simulink model "MomentEquation"  (R2024b)
settings: Solver=ode4  StartTime=0.0  StopTime=10  FixedStep=0.001  RelTol=1e-3
PreLoadFcn:
  | run UAVProperty
values from neighbouring files (symbols this model uses):
  I = [Ixx Ixy Ixz ... (first row only)    [UAVProperty.m]    (also in UnmannedAerialVehicle.m)
libraries: simulink x3, shared6dof x1, matrix_library x1
settings Model: Creator=LocoalKOH  LastModifiedBy=LocoalKOH

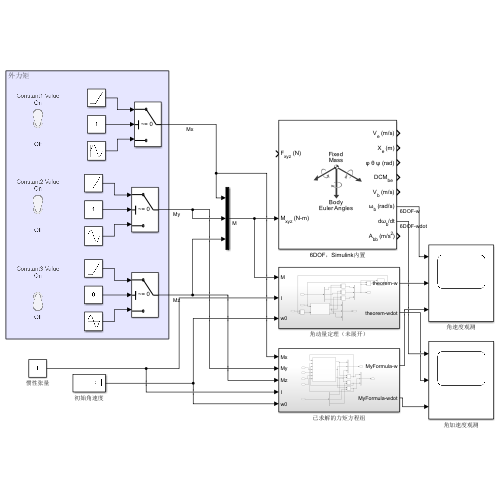
[thumbnail: Simulink's stored preview of the top-level diagram]
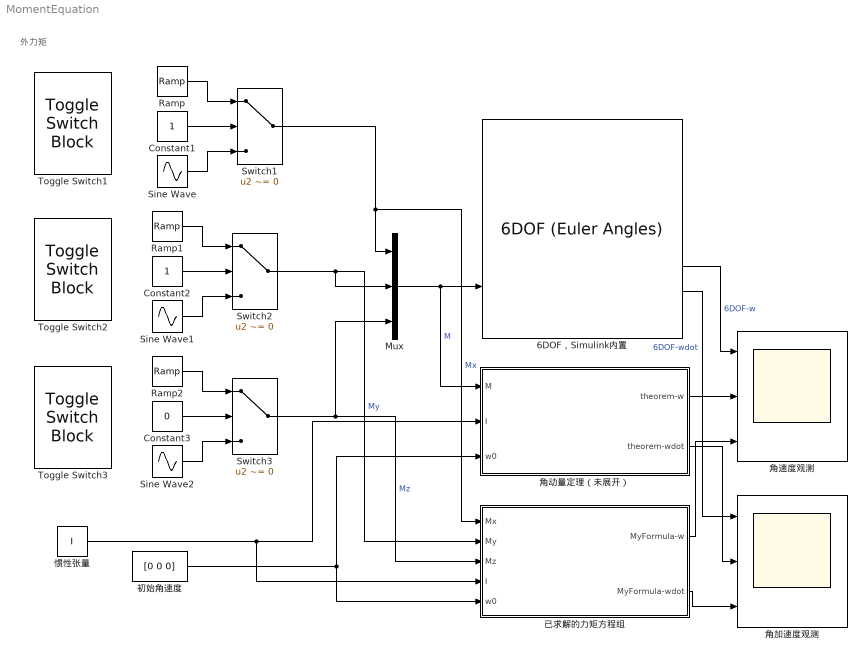
== system MomentEquation ==
  note: 外力矩
  6DOF，Simulink内置 : shared6dof/6DOF (Euler Angles)  units=Metric (MKS)  mtype=Fixed  rep=Euler Angles  xme_0=[0 0 0]  Vm_0=[0 0 0]  eul_0=[0 0 0]  pm_0=[0 0 0]  mass_0=Mass  mass_e=0.5  mass_f=2.0  inertia=I  inertia_e=eye(3)  inertia_f=2*eye(3)  k_quat=1.0  vre_flag=on  abi_flag=off  aMode=0  xme_statename=''  Vm_statename=''  eul_statename=''  quat_statename=''  pm_statename=''  mass_statename=''
  Constant1 : Constant
  Constant2 : Constant
  Constant3 : Constant  Value=0
  Mux : Mux  Inputs=3
  Ramp : simulink/Sources/Ramp  slope=5  start=0  InitialOutput=0
  Ramp1 : simulink/Sources/Ramp  slope=6000  start=0  InitialOutput=0
  Ramp2 : simulink/Sources/Ramp  slope=20  start=0  InitialOutput=8
  Sine Wave : Sin  SampleTime=0
  Sine Wave1 : Sin  SampleTime=0
  Sine Wave2 : Sin  Amplitude=7  Frequency=5  Phase=8  SampleTime=0
  Switch1 : Switch  Criteria=u2 ~= 0  SaturateOnIntegerOverflow=off  InputSameDT=off
  Switch2 : Switch  Criteria=u2 ~= 0  SaturateOnIntegerOverflow=off  InputSameDT=off
  Switch3 : Switch  Criteria=u2 ~= 0  SaturateOnIntegerOverflow=off  InputSameDT=off
  Toggle Switch1 : ToggleSwitchBlock
      settings: Values={{'Off', 'On'}, [0 1]}
  Toggle Switch2 : ToggleSwitchBlock
      settings: Values={{'Off', 'On'}, [0 1]}
  Toggle Switch3 : ToggleSwitchBlock
      settings: Values={{'Off', 'On'}, [0 1]}
  初始角速度 : Constant  Value=[0 0 0]  VectorParams1D=off
  已求解的力矩方程组 : Subsystem
  惯性张量 : Constant  Value=I  VectorParams1D=off  SampleTime=Inf
  角加速度观测 : Scope  NumInputPorts=3
  角动量定理（未展开） : Subsystem
  角速度观测 : Scope  NumInputPorts=3
  wires:
  Switch3/1 -> 已求解的力矩方程组/3(Mz), Mux/3  "Mz"
  Switch2/1 -> 已求解的力矩方程组/2(My), Mux/2  "My"
  惯性张量/1 -> 角动量定理（未展开）/2(I), 已求解的力矩方程组/4(I)
  Mux/1 -> 6DOF，Simulink内置/2, 角动量定理（未展开）/1(M)  "M"
  Switch1/1 -> 已求解的力矩方程组/1(Mx), Mux/1  "Mx"
  已求解的力矩方程组/1(MyFormula-w) -> 角速度观测/3
  初始角速度/1 -> 已求解的力矩方程组/5(w0), 角动量定理（未展开）/3(w0)
  6DOF，Simulink内置/7 -> 角加速度观测/1  "6DOF-wdot"
  6DOF，Simulink内置/6 -> 角速度观测/1  "6DOF-w"
  角动量定理（未展开）/1(theorem-w) -> 角速度观测/2
  角动量定理（未展开）/2(theorem-wdot) -> 角加速度观测/2
  已求解的力矩方程组/2(MyFormula-wdot) -> 角加速度观测/3
  Sine Wave1/1 -> Switch2/3
  Sine Wave2/1 -> Switch3/3
  Sine Wave/1 -> Switch1/3
  Constant3/1 -> Switch3/2
  Constant1/1 -> Switch1/2
  Constant2/1 -> Switch2/2
  Ramp2/1 -> Switch3/1
  Ramp/1 -> Switch1/1
  Ramp1/1 -> Switch2/1

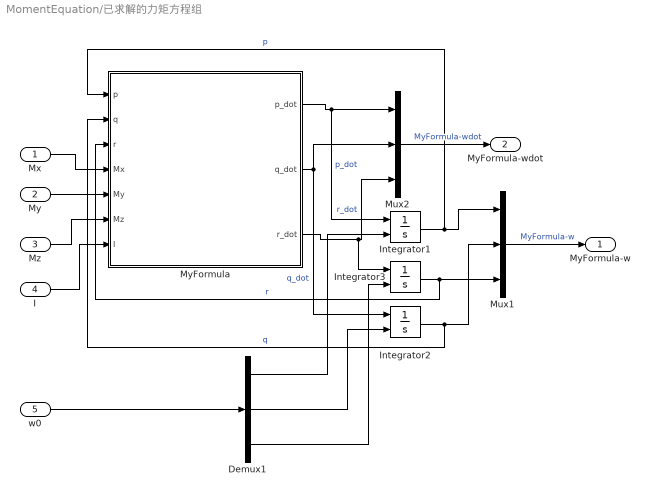
== system MomentEquation/已求解的力矩方程组 ==
  Mx : Inport
  My : Inport  Port=2
  Mz : Inport  Port=3
  I : Inport  Port=4
  w0 : Inport  Port=5
  Demux1 : Demux  Outputs=3
  Integrator1 : Integrator  InitialConditionSource=external
  Integrator2 : Integrator  InitialConditionSource=external
  Integrator3 : Integrator  InitialConditionSource=external
  Mux1 : Mux  Inputs=3
  Mux2 : Mux  Inputs=3
  MyFormula : MATLAB Function  TreatAsAtomicUnit=on
  MyFormula-w : Outport
  MyFormula-wdot : Outport  Port=2
  wires:
  Mx/1 -> MyFormula/4(Mx)
  My/1 -> MyFormula/5(My)
  Mz/1 -> MyFormula/6(Mz)
  I/1 -> MyFormula/7(I)
  MyFormula/3(r_dot) -> Mux2/3, Integrator3/1  "r_dot"
  MyFormula/2(q_dot) -> Integrator2/1, Mux2/2  "q_dot"
  MyFormula/1(p_dot) -> Mux2/1, Integrator1/1  "p_dot"
  w0/1 -> Demux1/1
  Demux1/1 -> Integrator1/2
  Demux1/2 -> Integrator2/2
  Demux1/3 -> Integrator3/2
  Mux2/1 -> MyFormula-wdot/1  "MyFormula-wdot"
  Integrator2/1 -> MyFormula/2(q), Mux1/2  "q"
  Integrator3/1 -> MyFormula/3(r), Mux1/3  "r"
  Integrator1/1 -> MyFormula/1(p), Mux1/1  "p"
  Mux1/1 -> MyFormula-w/1  "MyFormula-w"

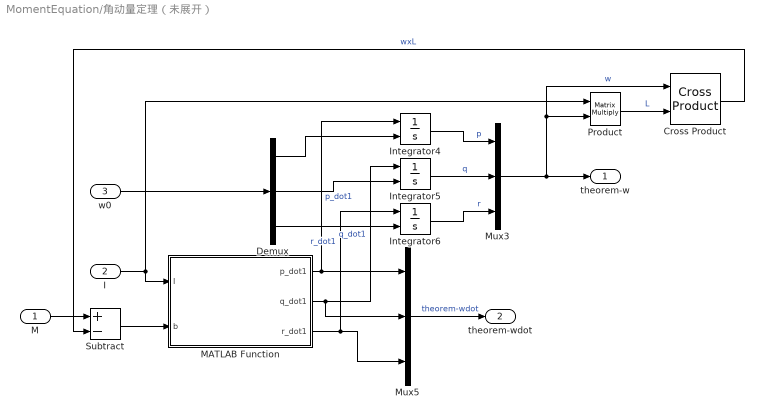
== system MomentEquation/角动量定理（未展开） ==
  M : Inport
  I : Inport  Port=2
  w0 : Inport  Port=3
  Cross Product : matrix_library/Cross Product
  Demux : Demux  Outputs=3
  Integrator4 : Integrator  InitialConditionSource=external
  Integrator5 : Integrator  InitialConditionSource=external
  Integrator6 : Integrator  InitialConditionSource=external
  MATLAB Function : MATLAB Function  TreatAsAtomicUnit=on
  Mux3 : Mux  Inputs=3
  Mux5 : Mux  Inputs=3
  Product : Product  Multiplication=Matrix(*)
  Subtract : Sum  Inputs=+-
  theorem-w : Outport
  theorem-wdot : Outport  Port=2
  wires:
  I/1 -> Product/1, MATLAB Function/1(I)
  M/1 -> Subtract/1
  w0/1 -> Demux/1
  Subtract/1 -> MATLAB Function/2(b)
  Demux/3 -> Integrator6/2
  Cross Product/1 -> Subtract/2  "wxL"
  Demux/2 -> Integrator5/2
  Demux/1 -> Integrator4/2
  MATLAB Function/1(p_dot1) -> Integrator4/1, Mux5/1  "p_dot1"
  MATLAB Function/2(q_dot1) -> Integrator5/1, Mux5/2  "q_dot1"
  MATLAB Function/3(r_dot1) -> Integrator6/1, Mux5/3  "r_dot1"
  Integrator4/1 -> Mux3/1  "p"
  Integrator6/1 -> Mux3/3  "r"
  Integrator5/1 -> Mux3/2  "q"
  Mux5/1 -> theorem-wdot/1  "theorem-wdot"
  Mux3/1 -> Cross Product/1, Product/2, theorem-w/1  "w"
  Product/1 -> Cross Product/2  "L"

== matlab function MomentEquation/角动量定理（未展开）/MATLAB Function ==
  data: I input; p_dot1 output; b input; q_dot1 output; r_dot1 output
function [p_dot1,q_dot1,r_dot1] = SolveEquations(I,b)

x = I \ b;
p_dot1 = x(1);
q_dot1 = x(2);
r_dot1 = x(3);
end

== matlab function MomentEquation/已求解的力矩方程组/MyFormula ==
  data: p input; q input; r input; Mx input; p_dot output; q_dot output; r_dot output; My input; Mz input; I input
function [p_dot,q_dot,r_dot] = Moment(p,q,r,Mx,My,Mz,I)
Ixx = I(1,1);   Iyy = I(2,2);   Izz = I(3,3);
Ixy = I(1,2);   Ixy = I(2,1);
Iyz = I(2,3);   Iyz = I(3,2);
Ixz = I(1,3);   Ixz = I(3,1);

Sigma = - Izz*Ixy^2 + 2*Ixy*Ixz*Iyz - Iyy*Ixz^2 - Ixx*Iyz^2 + Ixx*Iyy*Izz;

c1 = Iyy*Izz - Iyz^2;
c2 = Ixz*Iyz - Ixy*Izz;
c3 = Ixy*Iyz - Ixz*Iyy;
c4 = Ixz^2*Iyz - Ixy^2*Iyz + Ixy*Ixz*Iyy - Ixy*Ixz*Izz;
c5 = Ixy^2*Iyz - Ixz*Iyy*Ixy + Iyz^3 - Iyy*Izz*Iyz;
c6 = - Ixz^2*Iyz + Ixy*Izz*Ixz - Iyz^3 + Iyy*Izz*Iyz;
c7 = Ixz*Iyy^2 + 2*Ixz*Iyz^2 + Ixx*Ixy*Iyz - Ixx*Ixz*Iyy - Ixy*Iyy*Iyz - Ixy*Iyz*Izz - Ixz*Iyy*Izz;
c8 = Ixy^2*Izz - Ixz^2*Iyy + Iyy^2*Izz - Iyy*Iyz^2 - Iyy*Izz^2 + Iyz^2*Izz;
c9 = Ixx*Ixy*Izz - Ixy*Izz^2 - Ixx*Ixz*Iyz - 2*Ixy*Iyz^2 + Ixz*Iyy*Iyz + Ixy*Iyy*Izz + Ixz*Iyz*Izz;

p_dot = ...
    (c1/Sigma)*Mx ...
    + (c2/Sigma)*My ...
    + (c3/Sigma)*Mz ...
    + (c4/Sigma)*p^2 ...
    + (c5/Sigma)*q^2 ...
    + (c6/Sigma)*r^2 ...
    + (c7/Sigma)*p*q ...
    + (c8/Sigma)*q*r ...
    + (c9/Sigma)*p*r;

c10 = Ixz*Iyz - Ixy*Izz;
c11 = Ixx*Izz - Ixz^2;
c12 = Ixy*Ixz - Ixx*Iyz;
c13 = - Ixy^2*Ixz + Ixx*Iyz*Ixy - Ixz^3 + Ixx*Izz*Ixz;
c14 = Ixy^2*Ixz - Ixz*Iyz^2 - Ixx*Ixy*Iyz + Ixy*Iyz*Izz;
c15 = Ixz^3 + Ixz*Iyz^2 - Ixx*Izz*Ixz - Ixy*Izz*Iyz;
c16 = Ixx*Ixy*Ixz - 2*Ixz^2*Iyz - Ixx^2*Iyz - Ixy*Ixz*Iyy + Ixx*Iyy*Iyz + Ixy*Ixz*Izz + Ixx*Iyz*Izz;
c17 = 2*Ixy*Ixz^2 + Ixy*Izz^2 - Ixx*Ixz*Iyz - Ixx*Ixy*Izz + Ixz*Iyy*Iyz - Ixy*Iyy*Izz - Ixz*Iyz*Izz;
c18 = - Ixx^2*Izz + Ixx*Ixz^2 + Ixx*Iyz^2 + Ixx*Izz^2 - Ixy^2*Izz - Ixz^2*Izz;

q_dot = ...
    (c10/Sigma)*Mx ...
    + (c11/Sigma)*My ...
    + (c12/Sigma)*Mz ...
    + (c13/Sigma)*p^2 ...
    + (c14/Sigma)*q^2 ...
    + (c15/Sigma)*r^2 ...
    + (c16/Sigma)*p*q ...
    + (c17/Sigma)*q*r ...
    + (c18/Sigma)*p*r;

c19 = Ixy*Iyz - Ixz*Iyy;
c20 = Ixy*Ixz - Ixx*Iyz;
c21 = Ixx*Iyy - Ixy^2;
c22 = Ixy^3 + Ixy*Ixz^2 - Ixx*Iyy*Ixy - Ixx*Iyz*Ixz;
c23 = - Ixy^3 - Ixy*Iyz^2 + Ixx*Iyy*Ixy + Ixz*Iyy*Iyz;
c24 = Ixy*Iyz^2 - Ixy*Ixz^2 + Ixx*Ixz*Iyz - Ixz*Iyy*Iyz;
c25 = Ixx^2*Iyy - Ixx*Ixy^2 - Ixx*Iyy^2 - Ixx*Iyz^2 + Ixy^2*Iyy + Ixz^2*Iyy;
c26 = Ixx*Ixy*Iyz - Ixz*Iyy^2 - 2*Ixy^2*Ixz + Ixx*Ixz*Iyy + Ixy*Iyy*Iyz - Ixy*Iyz*Izz + Ixz*Iyy*Izz;
c27 = Ixx^2*Iyz + 2*Ixy^2*Iyz - Ixx*Ixy*Ixz - Ixy*Ixz*Iyy - Ixx*Iyy*Iyz + Ixy*Ixz*Izz - Ixx*Iyz*Izz;

r_dot = ...
    (c19/Sigma)*Mx ...
    + (c20/Sigma)*My ...
    + (c21/Sigma)*Mz ...
    + (c22/Sigma)*p^2 ...
    + (c23/Sigma)*q^2 ...
    + (c24/Sigma)*r^2 ...
    + (c25/Sigma)*p*q ...
    + (c26/Sigma)*q*r ...
    + (c27/Sigma)*p*r;

end
